simulink model "DCDC_PSFB_buck_boost_Converter"  (R2024b)
settings: Solver=FixedStepDiscrete  StartTime=0.0  StopTime=0.5  FixedStep=1e-6
values from neighbouring files (symbols this model uses):
  fs = 140e3    (= 140000)    [PSFB_Calculation_Code.m]    (also in PSFB_DCDC_Conveter_Calculation.m)
  N = Vout_max/Vin    (= 33.9583333333)    [PSFB_Calculation_Code.m]    (also in PSFB_DCDC_Conveter_Calculation.m = 0.03125)
  R_load = (Vout^2) / Pout    (= 116.363636364)    [PSFB_Calculation_Code.m]    (also in PSFB_DCDC_Conveter_Calculation.m = 0.104727272727)
  Vin = 24    [PSFB_Calculation_Code.m]    (also in PSFB_DCDC_Conveter_Calculation.m = 800)
  Vout = 800    [PSFB_Calculation_Code.m]    (also in PSFB_DCDC_Conveter_Calculation.m = 24; PSFB_Result_Plot_Code.m = Vout_sig.Data(:))
libraries: spsMosfetLib x8, spsDiodeLib x4, spsSeriesRLCBranchLib x4, spsCurrentMeasurementLib x3, spsVoltageMeasurementLib x3, spsGroundLib x1, spsDCVoltageSourceLib x1, slpidlib x1, spsVariableRatioTransformerLib x1, sps_lib x1
settings Model: Creator=SUDHAK1  LastModifiedBy=SUDHAK1

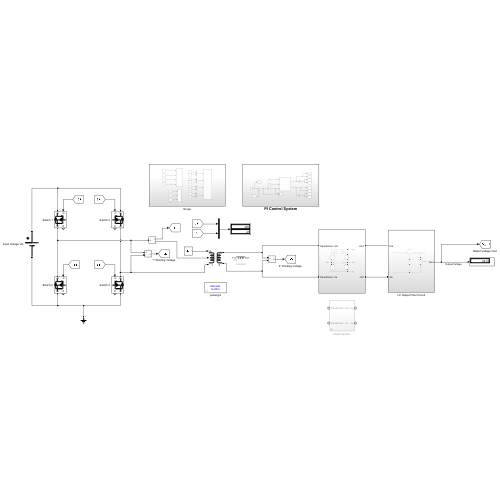
[thumbnail: Simulink's stored preview of the top-level diagram]
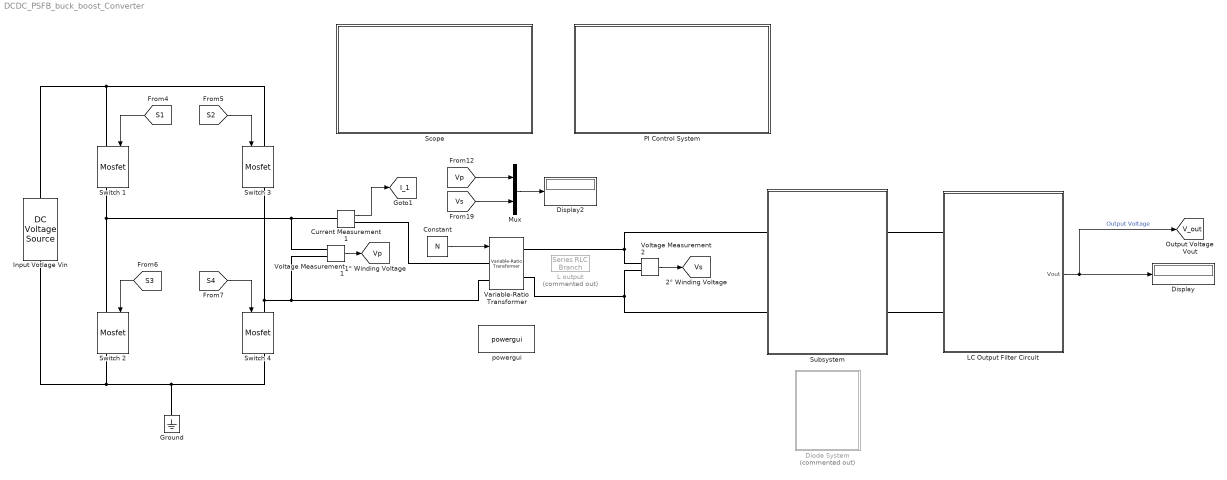
== system DCDC_PSFB_buck_boost_Converter ==
  Constant : Constant  Value=N
  Current Measurement1 : spsCurrentMeasurementLib/Current Measurement  PhasorSimulation=off  OutputType=Complex  PSBequivalent=0
  Diode System : Subsystem  Commented=on
  Display : Display
  Display2 : Display
  Ground : spsGroundLib/Ground  LConnTagsString=a
  Input Votlage Vin : spsDCVoltageSourceLib/DC Voltage Source  Amplitude=Vin  Measurements=Voltage
  L output : spsSeriesRLCBranchLib/Series RLC Branch  Commented=on  LConnTagsString=__new0  RConnTagsString=__new0  BranchType=L  Resistance=1  Inductance=1e-3  SetiL0=off  InitialCurrent=0  Capacitance=1e-6  Setx0=off  InitialVoltage=0  Measurements=None
  LC Output Filter Circuit : Subsystem
  Mux : Mux  Inputs=2
  PI Control System : Subsystem
  Scope : Subsystem
  Subsystem : Subsystem
  Switch {1..4} (4 alike) : spsMosfetLib/Mosfet  Ron=0.001  Lon=0  Rd=0.001  Vfd=0  IC=0  Rs=1e5  Cs=inf  Measurements=on
  Variable-Ratio Transformer : spsVariableRatioTransformerLib/Variable-Ratio Transformer
      settings: LibrarySourceBlock=|
      | sps_lib/Passives/Variable-Ratio
      | Transformer
  Voltage Measurement1 : spsVoltageMeasurementLib/Voltage Measurement  PhasorSimulation=off  OutputType=Complex  PSBequivalent=0
  Voltage Measurement2 : spsVoltageMeasurementLib/Voltage Measurement  PhasorSimulation=off  OutputType=Complex  PSBequivalent=0
  powergui : sps_lib/powergui  Priority=1  SimulationMode=Discrete  SampleTime=1e-6  frequency=60  Iterations=50  frequencyindice=0  Pbase=100e6  ErrMax=1e-4  UnitsV=kV  UnitsW=MW  buscounter=0  FunctionMessages=off  echomessages=off  EnableUseOfTLC=off  CurrentSourceSwitches=off  DisableSnubberDevices=off  DisableRonSwitches=off  DisableVfSwitches=off  DisplayEquations=off  AutomaticDiscreteSolvers=off  SolverType=Tustin/Backward Euler (TBE)  Interpol=off  ExternalGateDelay=off  methode=off  Ts=100  x0status=blocks  SPID=on  SwTol=0  HookPort=off  NonlinearTolerance=1e-4  nMaxIteration=100  ContinueOnMaxIteration=off  RestoreLinks=warning  ResistiveCurrentMeasurement=off  Frange=[0:2:500]  Ylog=off  Xlog=on  ShowGrid=off  save=off  variable=ZData  structure=0  ZoomFFT=off  StartTime=0.0  cycles=1  DisplayStyle=1  fundamental=60  FreqAxis=off  MaxFrequency=1000  frequencyindicesteady=1  RmsSteady=1  display=off
  tag scope: I_1=global, V_out=global, Vp=global, Vs=global
  wires:
  [S1] -> Switch 1/1
  Voltage Measurement1/1 -> [Vp]
  Current Measurement1/1 -> [I_1]
  Voltage Measurement2/1 -> [Vs]
  [S4] -> Switch 4/1
  LC Output Filter Circuit/1(Vout) -> [V_out], Display/1  "Output Voltage"
  [Vp] -> Mux/1
  [Vs] -> Mux/2
  Mux/1 -> Display2/1
  [S3] -> Switch 2/1
  [S2] -> Switch 3/1
  Constant/1 -> Variable-Ratio Transformer/1
  connections:
  Switch 2/RConn1 -- Input Votlage Vin/LConn1 -- Ground/LConn1 -- Switch 4/RConn1
  Switch 3/RConn1 -- Voltage Measurement1/LConn2 -- Variable-Ratio Transformer/LConn2 -- Switch 4/LConn1
  Switch 1/LConn1 -- Input Votlage Vin/RConn1 -- Switch 3/LConn1
  Voltage Measurement2/LConn2 -- Subsystem/LConn2 -- Variable-Ratio Transformer/RConn2
  Subsystem/RConn1 -- LC Output Filter Circuit/LConn1
  Subsystem/RConn2 -- LC Output Filter Circuit/LConn2
  Voltage Measurement2/LConn1 -- Variable-Ratio Transformer/RConn1 -- Subsystem/LConn1
  Switch 1/RConn1 -- Switch 2/LConn1 -- Current Measurement1/LConn1 -- Voltage Measurement1/LConn1
  Current Measurement1/RConn1 -- Variable-Ratio Transformer/LConn1

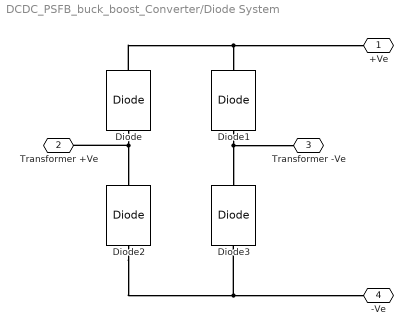
== system DCDC_PSFB_buck_boost_Converter/Diode System ==
  Diode{,1..3} (4 alike) : spsDiodeLib/Diode  Ron=0.001  Lon=0  Vf=0.8  IC=0  UseSnubber=0  Rs=500  Cs=250e-9  Measurements=off
  +Ve : PMIOPort  Side=Right
  Transformer +Ve : PMIOPort  Port=2  Side=Left
  Transformer -Ve : PMIOPort  Port=3  Side=Left
  -Ve : PMIOPort  Port=4  Side=Right
  connections:
  Diode/RConn1 -- Diode1/RConn1 -- +Ve/RConn1
  Diode/LConn1 -- Transformer +Ve/RConn1 -- Diode2/RConn1
  Diode2/LConn1 -- -Ve/RConn1 -- Diode3/LConn1
  Diode1/LConn1 -- Diode3/RConn1 -- Transformer -Ve/RConn1

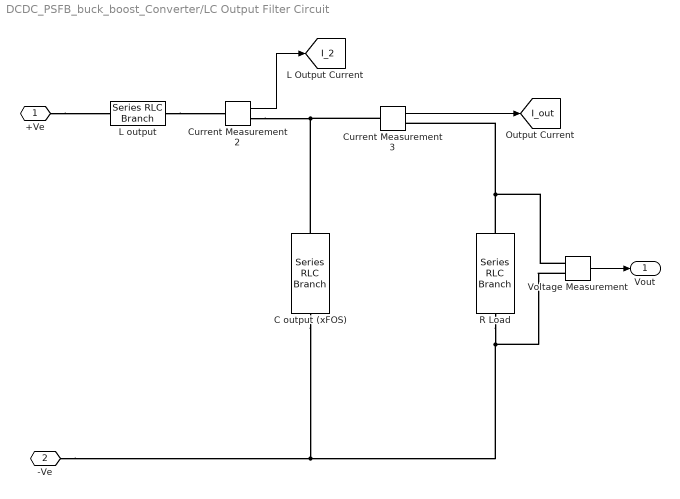
== system DCDC_PSFB_buck_boost_Converter/LC Output Filter Circuit ==
  C output (xFOS) : spsSeriesRLCBranchLib/Series RLC Branch  LConnTagsString=__new0  RConnTagsString=__new0  BranchType=C  Resistance=1  Inductance=7.8e-7  SetiL0=off  InitialCurrent=0  Capacitance=3e-3  Setx0=off  InitialVoltage=0  Measurements=None
  Current Measurement2 : spsCurrentMeasurementLib/Current Measurement  PhasorSimulation=off  OutputType=Complex  PSBequivalent=0
  Current Measurement3 : spsCurrentMeasurementLib/Current Measurement  PhasorSimulation=off  OutputType=Complex  PSBequivalent=0
  L output : spsSeriesRLCBranchLib/Series RLC Branch  LConnTagsString=__new0  RConnTagsString=__new0  BranchType=L  Resistance=1  Inductance=5e-3  SetiL0=off  InitialCurrent=0  Capacitance=1e-6  Setx0=off  InitialVoltage=0  Measurements=None
  R Load : spsSeriesRLCBranchLib/Series RLC Branch  LConnTagsString=__new0  RConnTagsString=__new0  BranchType=R  Resistance=R_load  Inductance=1e-3  SetiL0=off  InitialCurrent=0  Capacitance=1e-6  Setx0=off  InitialVoltage=0  Measurements=None
  Voltage Measurement : spsVoltageMeasurementLib/Voltage Measurement  PhasorSimulation=off  OutputType=Complex  PSBequivalent=0
  +Ve : PMIOPort  Side=Left
  -Ve : PMIOPort  Port=2  Side=Left
  Vout : Outport
  tag scope: I_2=global, I_out=global
  wires:
  Current Measurement3/1 -> [I_out]
  Current Measurement2/1 -> [I_2]
  Voltage Measurement/1 -> Vout/1
  connections:
  R Load/LConn1 -- Voltage Measurement/LConn1 -- Current Measurement3/RConn1
  Voltage Measurement/LConn2 -- R Load/RConn1 -- -Ve/RConn1 -- C output (xFOS)/RConn1
  L output/RConn1 -- Current Measurement2/LConn1
  C output (xFOS)/LConn1 -- Current Measurement2/RConn1 -- Current Measurement3/LConn1
  +Ve/RConn1 -- L output/LConn1

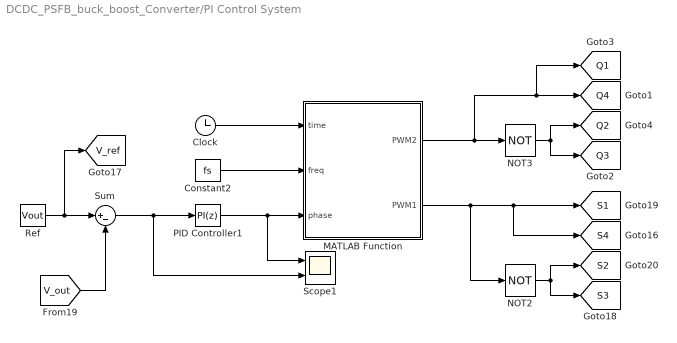
== system DCDC_PSFB_buck_boost_Converter/PI Control System ==
  Clock : Clock
  Constant2 : Constant  Value=fs
  MATLAB Function : MATLAB Function  TreatAsAtomicUnit=on
  NOT2 : Logic  Operator=NOT  IconShape=distinctive  AllPortsSameDT=off  OutDataTypeStr=boolean
  NOT3 : Logic  Operator=NOT  IconShape=distinctive  AllPortsSameDT=off  OutDataTypeStr=boolean
  PID Controller1 : slpidlib/PID Controller  Controller=PI  Form=Parallel  TimeDomain=Discrete-time  UseExternalTs=off  SampleTime=-1  IntegratorMethod=Forward Euler  FilterMethod=Forward Euler  ControllerParametersSource=internal  P=0.00001  I=0.01  UseKiTs=off  D=0  UseExternalDerivativeSource=off  N=100  UseFilter=on  TunerSelectOption=Transfer Function Based (PID Tuner App)  InitialConditionSource=internal  InitialConditionForIntegrator=0  InitialConditionForFilter=0  DifferentiatorICPrevScaledInput=0  ExternalReset=none  TrackingMode=off  Kt=1  LimitOutput=on  SatLimitsSource=internal  UpperSaturationLimit=180  LowerSaturationLimit=0  LinearizeAsGain=on  AntiWindupMode=none  Kb=1  LimitIntegrator=off  UpperIntegratorSaturationLimit=inf  LowerIntegratorSaturationLimit=-inf  POutMin=[]  POutMax=[]  IOutMin=[]  IOutMax=[]  DOutMin=[]  DOutMax=[]  NOutMin=[]  NOutMax=[]  SumOutMin=[]  SumOutMax=[]  SaturationOutMin=[]  SaturationOutMax=[]  PParamMin=[]  PParamMax=[]  IParamMin=[]  IParamMax=[]  DParamMin=[]  DParamMax=[]  NParamMin=[]  NParamMax=[]  KbParamMin=[]  KbParamMax=[]  KtParamMin=[]  KtParamMax=[]  KbOutMin=[]  KbOutMax=[]  KtOutMin=[]  KtOutMax=[]  IntegratorOutMin=[]  IntegratorOutMax=[]  FilterOutMin=[]  FilterOutMax=[]  SumI1OutMin=[]  SumI1OutMax=[]  SumI2OutMin=[]  SumI2OutMax=[]  SumI3OutMin=[]  SumI3OutMax=[]  SumI4OutMin=[]  SumI4OutMax=[]  SumDOutMin=[]  SumDOutMax=[]  DifferentiatorOutMin=[]  DifferentiatorOutMax=[]  FilterDiffOutCoefMin=[]  FilterDiffOutCoefMax=[]  ReciprocalOutMin=[]  ReciprocalOutMax=[]  SumDenOutMin=[]  SumDenOutMax=[]  SumNumOutMin=[]  SumNumOutMax=[]  DivideOutMin=[]  DivideOutMax=[]  UdiffTsProdOutMin=[]  UdiffTsProdOutMax=[]  NTsProdOutMin=[]  NTsProdOutMax=[]  UintegralTsProdOutMin=[]  UintegralTsProdOutMax=[]  UngainTsProdOutMin=[]  UngainTsProdOutMax=[]  ClampingZeroOutDataTypeStr=Inherit: Inherit via back propagation  ClampingZeroOutMin=[]  ClampingZeroOutMax=[]  FilterDenConstantOutDataTypeStr=Inherit: Inherit via back propagation  FilterDenConstantOutMin=[]  FilterDenConstantOutMax=[]  PCopyOutDataTypeStr=Inherit: Inherit via back propagation  PCopyOutMin=[]  PCopyOutMax=[]  NCopyOutDataTypeStr=Inherit: Inherit via back propagation  NCopyOutMin=[]  NCopyOutMax=[]  IntegratorContinuousStateAttributes=''  IntegratorStateMustResolveToSignalObject=off  IntegratorRTWStateStorageClass=Auto  FilterContinuousStateAttributes=''  FilterStateMustResolveToSignalObject=off  FilterRTWStateStorageClass=Auto  ParallelPVariant=InternalParameters  IdealPVariant=Disabled  IVariant=InternalParameters  DVariant=Disabled  IntegratorVariant=Discrete  SatVariant=Enabled  AWVariant=Passthrough  PCopyVariant=Disabled  TRVariant=Disabled  FdbkBlocksVariant=Forward  IdealPFdbkVariant=Disabled  SatFdbkVariant=Disabled  DerivativeFilterVariant=Disabled  NVariant=Disabled  NCopyVariant=Disabled_SignalSpec  FilterICVariant=Disabled  IntegratorICVariant=InternalICs  ExternalResetVariant=Disabled  TRSumVariant=Passthrough  SumFdbkVariant=Disabled  SumVariant=Sum_PI  TsampFilterVariant=InternalTs  TsampNgainVariant=Passthrough  TsampIntegralVariant=Disabled_SignalSpec  ExternalSaturationOutDataTypeStr=Inherit: Same as second input  DerivativeSourceVariant=Disabled  PreIntVariant=InternalPreInt
  Ref : Constant  Value=Vout
  Scope1 : Scope  NumInputPorts=2
  Sum : Sum  Inputs=|+-
  tag scope: Q1=global, Q2=global, Q3=global, Q4=global, S1=global, S2=global, S3=global, S4=global, V_ref=global
  wires:
  Clock/1 -> MATLAB Function/1(time)
  [V_out] -> Sum/2
  Ref/1 -> [V_ref], Sum/1
  Constant2/1 -> MATLAB Function/2(freq)
  NOT3/1 -> [Q2], [Q3]
  NOT2/1 -> [S2], [S3]
  Sum/1 -> Scope1/2, PID Controller1/1
  MATLAB Function/2(PWM1) -> NOT2/1, [S4], [S1]
  MATLAB Function/1(PWM2) -> [Q1], [Q4], NOT3/1
  PID Controller1/1 -> Scope1/1, MATLAB Function/3(phase)

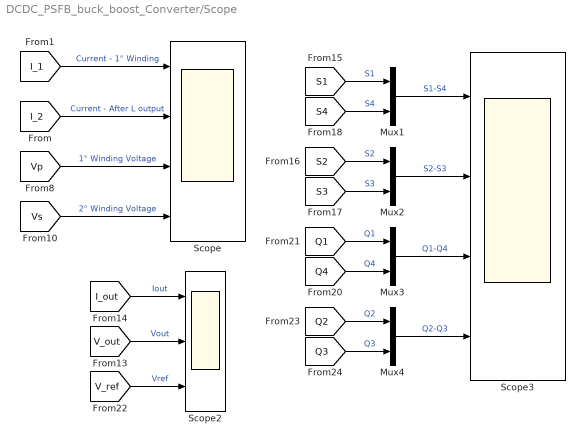
== system DCDC_PSFB_buck_boost_Converter/Scope ==
  Mux{1..4} (4 alike) : Mux  Inputs=2
  Scope : Scope  NumInputPorts=4
  Scope2 : Scope  NumInputPorts=3
  Scope3 : Scope  NumInputPorts=4
  wires:
  [Vp] -> Scope/3  "1° Winding Voltage"
  [I_out] -> Scope2/1  "Iout"
  [V_out] -> Scope2/2  "Vout"
  [I_2] -> Scope/2  "Current - After L output"
  [V_ref] -> Scope2/3  "Vref"
  [Vs] -> Scope/4  "2° Winding Voltage"
  [I_1] -> Scope/1  "Current - 1° Winding"
  Mux1/1 -> Scope3/1  "S1-S4"
  [S3] -> Mux2/2  "S3"
  Mux2/1 -> Scope3/2  "S2-S3"
  [S1] -> Mux1/1  "S1"
  [S4] -> Mux1/2  "S4"
  [S2] -> Mux2/1  "S2"
  Mux3/1 -> Scope3/3  "Q1-Q4"
  Mux4/1 -> Scope3/4  "Q2-Q3"
  [Q2] -> Mux4/1  "Q2"
  [Q3] -> Mux4/2  "Q3"
  [Q1] -> Mux3/1  "Q1"
  [Q4] -> Mux3/2  "Q4"

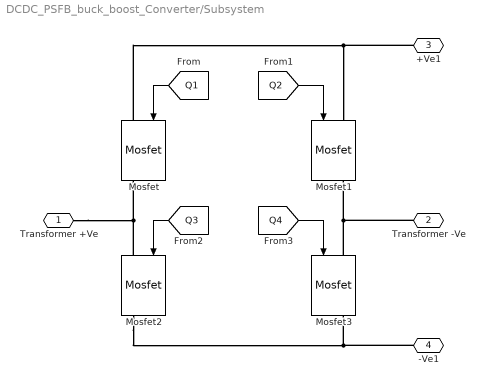
== system DCDC_PSFB_buck_boost_Converter/Subsystem ==
  Mosfet{,1..3} (4 alike) : spsMosfetLib/Mosfet  Ron=0.001  Lon=0  Rd=0.001  Vfd=0  IC=0  Rs=1e5  Cs=inf  Measurements=on
  Transformer +Ve : PMIOPort  Side=Left
  Transformer -Ve : PMIOPort  Port=2  Side=Left
  +Ve1 : PMIOPort  Port=3  Side=Right
  -Ve1 : PMIOPort  Port=4  Side=Right
  wires:
  [Q1] -> Mosfet/1
  [Q4] -> Mosfet3/1
  [Q3] -> Mosfet2/1
  [Q2] -> Mosfet1/1
  connections:
  +Ve1/RConn1 -- Mosfet1/LConn1 -- Mosfet/LConn1
  -Ve1/RConn1 -- Mosfet3/RConn1 -- Mosfet2/RConn1
  Mosfet3/LConn1 -- Mosfet1/RConn1 -- Transformer -Ve/RConn1
  Mosfet2/LConn1 -- Transformer +Ve/RConn1 -- Mosfet/RConn1

== matlab function DCDC_PSFB_buck_boost_Converter/PI Control System/MATLAB Function ==
  data: time input; PWM2 output; PWM1 output; freq input; phase input
function [PWM2,PWM1] = fcn(time,freq,phase)
Tswitching = 1/freq;
PWM1 = 0;
PWM2 = 0;

y1 = mod(time,Tswitching);

if y1 < Tswitching/2
    PWM1 = 1;
end  

t_phi = Tswitching*(phase/360);

y2=mod(time+t_phi,Tswitching);

if y2 < Tswitching/2
    PWM2 = 1;
end
